simulink model "SYS_CL_X_ref"  (R2026a)
settings: Solver=VariableStepAuto  StopTime=150.0
undefined symbols (not defined in the file): K_d_x_ref, K_p_x_ref
libraries: simulink x1, cstblocks_lti x1
settings Model: Creator=samuel  LastModifiedBy=samuel

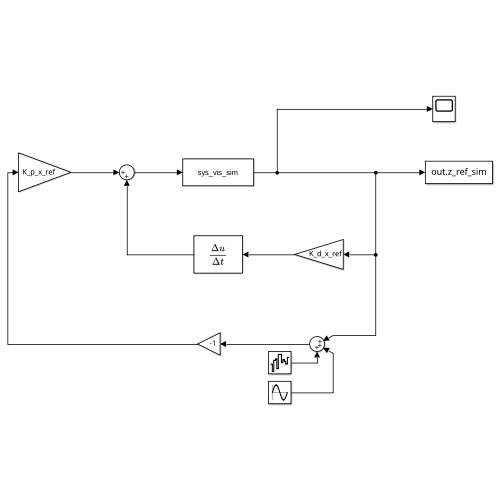
[thumbnail: Simulink's stored preview of the top-level diagram]
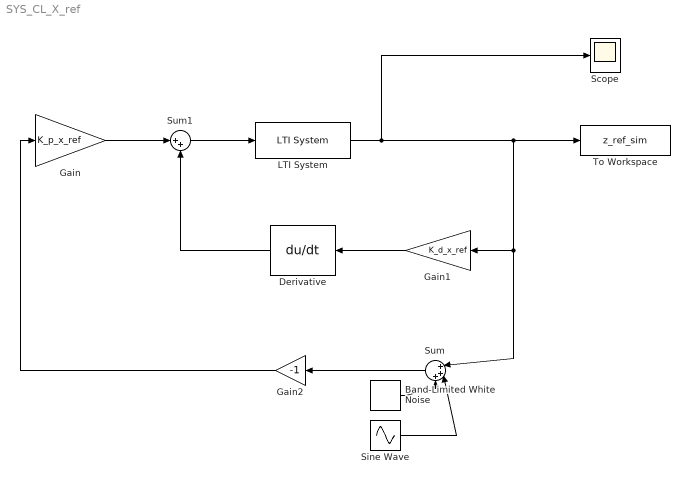
== system SYS_CL_X_ref ==
  Band-Limited White Noise : simulink/Sources/Band-Limited White Noise  Cov=[0.1]  Ts=0.1  seed=[23341]
  Derivative : Derivative
  Gain : Gain  Gain=K_p_x_ref
  Gain1 : Gain  Gain=K_d_x_ref
  Gain2 : Gain  Gain=-1
  LTI System : cstblocks_lti/LTI System  sys=sys_vis_sim  IC=[]  PadeOrder=0
      settings: LibrarySourceBlock=cstblocks/LTI System
  Scope : Scope
      settings: ActiveDisplayYMinimum=-0.54867833163319868  ActiveDisplayYMaximum=0.34946343259103735
  Sine Wave : Sin  Amplitude=10  SampleTime=0
  Sum : Sum  Inputs=|+++
  Sum1 : Sum  Inputs=|++
  To Workspace : ToWorkspace  VariableName=z_ref_sim  SaveFormat=Timeseries  SampleTime=-1
  wires:
  Sum1/1 -> LTI System/1
  Gain/1 -> Sum1/1
  Gain1/1 -> Derivative/1
  Derivative/1 -> Sum1/2
  LTI System/1 -> Sum/1, Gain1/1, To Workspace/1, Scope/1
  Gain2/1 -> Gain/1
  Sum/1 -> Gain2/1
  Sine Wave/1 -> Sum/2
  Band-Limited White Noise/1 -> Sum/3
